simulink model "crs_plant"  (R2026b)
settings: Solver=ode45  StopTime=80  FixedStep=Ts  EnableMultiTasking=on
model workspace (MAT data in the model file):
  Iei = 0.0219914882836
  converter_data = [0  137.465208994  2.232; 0.1  137.065019157  2.075; 0.2  135.864449646  1.975; 0.3  135.664354728  1.846; 0.4  137.565256453  1.72; 0.5  140.366585312  1.564; 0.6  145.268910814  1.409; 0.7  152.872517717  1.254; 0.8  162.9773111  1.096; 0.81  164.27792807  1.08; 0.82  166.178829795  1.061; 0.83  167.979684062  1.043; 0.84  170.080680706  1.028; 0.85  172.781962105  1.012; 0.86  175.383196045  1.002; 0.87  179.585189333  1.002; 0.88  183.587087703  1.001; 0.89  189.890077635  0.998; 0.9  197.693779455  0.999; 0.92  215.902417037  1.001; 0.94  244.515990379  1.002]
  emap = [-40  -44  -49  -53  -57  -61  -65  -70  -74  -78  -82; 215  117  85  66  44  29  10  -2  -13  -22  -32; 245  208  178  148  122  104  85  66  48  33  18; 264  260  241  219  193  167  152  133  119  96  85; 264  279  282  275  260  238  223  208  189  171  152; 267  290  293  297  290  275  260  256  234  212  193; 267  297  305  305  305  301  293  282  267  249  226; 267  301  308  312  319  323  319  316  297  279  253; 267  301  312  319  327  327  327  327  312  293  267; 267  301  312  319  327  334  334  334  319  305  275]
  nevec = [800 1200 1600 2000 2400 2800 3200 3600 4000 4400 4800]
  p0 = 0.07934
  p1 = 0.07934
  thvec = [0; 20; 30; 40; 50; 60; 70; 80; 90; 100]
  vehicledata = [3.23; 40; 0.3; 1; 50; 0]
undefined symbols (not defined in the file): downtab, downth, uptab, upth
settings Model: DataDictionary=crs_plantdic.sldd  SldvGeneratedHarnessModel=TestUnitModel=psui_cruise_control|  Creator=The MathWorks, Inc.  LastModifiedBy=The MathWorks, Inc.
settings DataIOCC: DSMLogging=off  ReturnWorkspaceOutputs=off  SaveFormat=StructureWithTime  SaveOutput=off  SaveTime=off  SignalLogging=off
settings OptimizationCC: BlockReduction=off  ConditionallyExecuteInputs=off  EfficientMapNaN2IntZero=off  LifeSpan=inf  UseDivisionForNetSlopeComputation=on
settings DebuggingCC: AllowSymbolicDim=off  ArithmeticOperatorsInVariantConditions=warning  InheritedTsInSrcMsg=none  SFExecutionAtInitializationDiag=none  SFNoUnconditionalDefaultTransitionDiag=warning  SFUnexpectedBacktrackingDiag=warning  SolverPrmCheckMsg=warning
settings HardwareCC: ProdEndianess=Unspecified  ProdHWDeviceType=32-bit Generic  ProdLargestAtomicFloat=None
settings ModelReferenceCC: PropagateSignalLabelsOutOfModel=off
settings SFSimCC: CustomCodeUndefinedFunction=UseInterfaceOnly  SimUseLocalCustomCode=off
settings RTWCC: DLArmComputeVersion=19.05  RTWUseLocalCustomCode=off
settings CodeAppCC: StateflowObjectComments=on
settings GRTTargetCC: TargetLangStandard=C89/C90 (ANSI)
settings ConfigComp: CovExternalEMLEnable=off  CovHTMLOptions=-sRT=1 -sVT=0 -aTS=1 -bRG=1 -bTC=0 -hTR=0 -nFC=0 -nFD=1 -scm=1 -bcm=1 -xEv=0 -xEM=0  CovMetricSettings=dcm  CovSFcnEnable=off  CovSaveCumulativeToWorkspaceVar=on  CovSaveSingleToWorkspaceVar=on  DVDefectChecker=off  DVDetectActiveLogic=on  DVHarnessSource=Signal Editor  DVSFcnSupport=off  DVTestSuiteOptimization=Auto

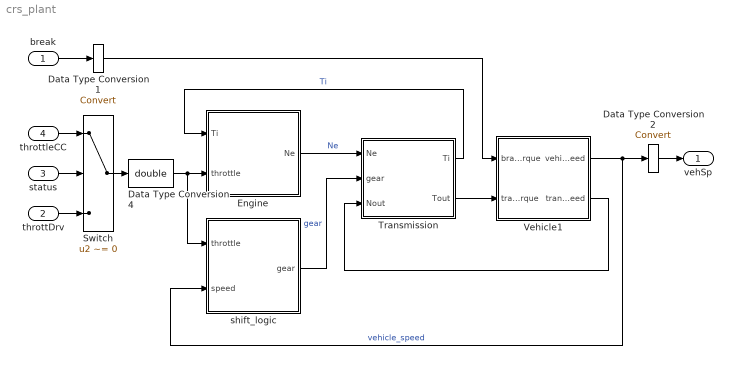
== system crs_plant ==
  break : Inport
  throttDrv : Inport  Port=2
  status : Inport  Port=3  OutDataTypeStr=boolean
  throttleCC : Inport  Port=4
  Data Type Conversion1 : DataTypeConversion  RequirementInfo="{}  %GIDa_0d5f0e68_fee1_41b5_819f_f27f813a37ce"  SaturateOnIntegerOverflow=off  RndMeth=Floor
  Data Type Conversion2 : DataTypeConversion  RequirementInfo="{}  %GIDa_2150bf92_ce46_40fc_a41f_e6b4de8980e5"  SaturateOnIntegerOverflow=off  RndMeth=Floor
  Data Type Conversion4 : DataTypeConversion  RequirementInfo="{}  %GIDa_40e403eb_4293_4261_b76c_ee9daf66d60d"  OutDataTypeStr=double  SaturateOnIntegerOverflow=off  RndMeth=Floor
  Engine : Subsystem
  Switch : Switch  RequirementInfo="{}  %GIDa_4750b5ac_669f_4708_bed6_ecccb1e59b59"  Criteria=u2 ~= 0  SaturateOnIntegerOverflow=off  InputSameDT=off
  Transmission : Subsystem
  Vehicle1 : Subsystem  mask(vehicle model){Rfd=vehicledata(1), rload0=vehicledata(2), rload2=vehicledata(3), Rw=vehicledata(4), Iv=vehicledata(5), N20=vehicledata(6)/vehicledata(4)*vehicledata(1)}
      mask prompts: Rfd "final drive ratio"; rload0 "drag friction at wheels"; rload2 "aerodynamic drag"; Rw "wheel radius"; Iv "vehicle inertia"; N20 "initial transmission output speed"
      mask help: vehicle dynamics: torque input from trans., outputs are input speed (transmission output) and vehicle speed
      mask Display: disp('Vehicle')
  shift_logic : Stateflow chart  TreatAsAtomicUnit=on  mask{TWAIT=2}
      mask prompts: TWAIT "Delay before gear change (tick)"
  vehSp : Outport  VectorParamsAs1DForOutWhenUnconnected=off
  wires:
  Data Type Conversion2/1 -> vehSp/1
  Data Type Conversion1/1 -> Vehicle1/1(brake torque)
  Data Type Conversion4/1 -> shift_logic/1(throttle), Engine/2(throttle)
  shift_logic/1(" gear") -> Transmission/2(gear)  "gear"
  Vehicle1/1(vehicle speed) -> shift_logic/2(speed), Data Type Conversion2/1  "vehicle_speed"
  break/1 -> Data Type Conversion1/1
  throttleCC/1 -> Switch/1
  Engine/1(Ne) -> Transmission/1(Ne)  "Ne"
  Transmission/1(Ti) -> Engine/1(Ti)  "Ti"
  status/1 -> Switch/2
  throttDrv/1 -> Switch/3
  Switch/1 -> Data Type Conversion4/1
  Transmission/2(Tout) -> Vehicle1/2(transmission output torque)
  Vehicle1/2(transmission output speed) -> Transmission/3(Nout)

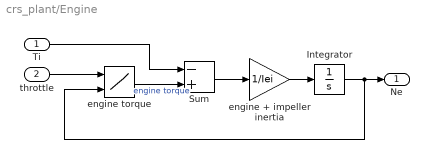
== system crs_plant/Engine ==
  Ti : Inport
  throttle : Inport  Port=2
  Integrator : Integrator  RequirementInfo="{}  %GIDa_40d16765_53ae_4488_8a68_ecbb2df0c680"  InitialCondition=1000  LimitOutput=on  UpperSaturationLimit=6000  LowerSaturationLimit=600  ZeroCross=off
  Sum : Sum  RequirementInfo="{}  %GIDa_1d505b5e_8a80_40cd_8acd_de2326c4a3eb"  Inputs=-+  InputSameDT=on  SaturateOnIntegerOverflow=on  OutDataTypeStr=Inherit: Same as first input
  engine torque : Lookup2D  RequirementInfo="{}  %GIDa_c9ecf741_2e32_444d_a0cd_5ec9da647599"  RowIndex=thvec*0.3  ColumnIndex=nevec  Table=emap  SaturateOnIntegerOverflow=off
  engine + impeller inertia : Gain  RequirementInfo="{}  %GIDa_fbb5ce3c_512e_47cd_b98c_f91ed20f1992"  Gain=1/Iei  SaturateOnIntegerOverflow=on  OutDataTypeStr=Inherit: Same as input  ParamDataTypeStr=Inherit: Same as input
  Ne : Outport  InitialOutput=0  VectorParamsAs1DForOutWhenUnconnected=off
  wires:
  engine torque/1 -> Sum/2  "engine torque"
  engine + impeller inertia/1 -> Integrator/1
  Sum/1 -> engine + impeller inertia/1
  Integrator/1 -> Ne/1, engine torque/2
  throttle/1 -> engine torque/1
  Ti/1 -> Sum/1

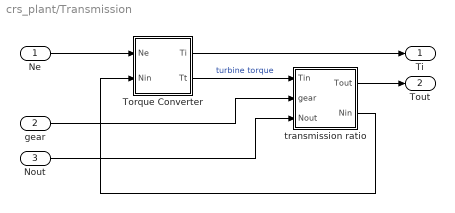
== system crs_plant/Transmission ==
  Ne : Inport
  gear : Inport  Port=2
  Nout : Inport  Port=3
  Torque Converter : Subsystem  mask(torque converter){speedratio=converter_data(:,1), Kfactor=converter_data(:,2), Torkratio=converter_data(:,3)}
      mask prompts: speedratio "speed ratio"; Kfactor "K factor"; Torkratio "torque ratio"
      mask help: torque converter
      mask Help: Torque converter input and output torques are computed as a function of the input and output speeds
      mask Display: plot([cos([90:10:450]*pi/180),.63*cos([90:10:450]*pi/180),.63*cos([90:10:240]*pi/180),cos([240:10:300]*pi/180),.63*cos([300]*pi/180)],[sin([90:10:450]*pi/180),.63*sin([90:10:450]*pi/180)+.1,.63*sin([90:10:240]*pi/180)+.1,sin([240:10:300]*pi/180),.63*sin([300]*pi/180)+.1])
  transmission ratio : Subsystem
  Ti : Outport  VectorParamsAs1DForOutWhenUnconnected=off
  Tout : Outport  Port=2  VectorParamsAs1DForOutWhenUnconnected=off
  wires:
  transmission ratio/1(Tout) -> Tout/1
  Torque Converter/1(Ti) -> Ti/1
  Nout/1 -> transmission ratio/3(Nout)
  gear/1 -> transmission ratio/2(gear)
  Ne/1 -> Torque Converter/1(Ne)
  transmission ratio/2(Nin) -> Torque Converter/2(Nin)
  Torque Converter/2(Tt) -> transmission ratio/1(Tin)  "turbine torque"

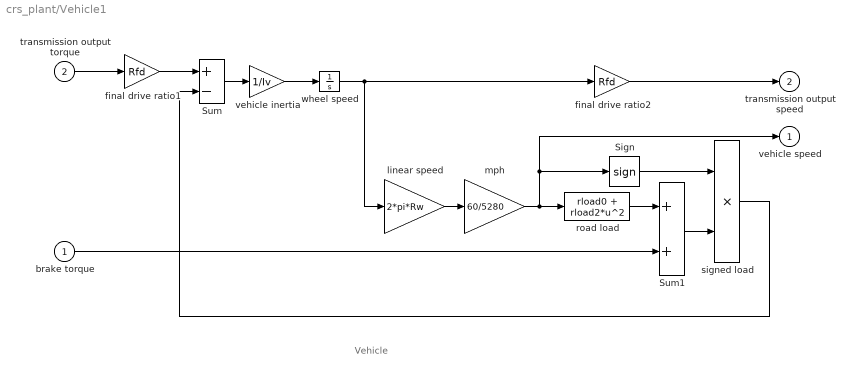
== system crs_plant/Vehicle1 ==
  note: Vehicle
  brake torque : Inport
  transmission output torque : Inport  Port=2
  Sign : Signum
  Sum : Sum  Inputs=+-  InputSameDT=on  SaturateOnIntegerOverflow=on  OutDataTypeStr=Inherit: Same as first input
  Sum1 : Sum  InputSameDT=on  SaturateOnIntegerOverflow=on  OutDataTypeStr=Inherit: Same as first input
  final drive ratio1 : Gain  Gain=Rfd  SaturateOnIntegerOverflow=on  OutDataTypeStr=Inherit: Same as input  ParamDataTypeStr=Inherit: Same as input
  final drive ratio2 : Gain  Gain=Rfd  SaturateOnIntegerOverflow=on  OutDataTypeStr=Inherit: Same as input  ParamDataTypeStr=Inherit: Same as input
  linear speed : Gain  Gain=2*pi*Rw  SaturateOnIntegerOverflow=on  OutDataTypeStr=Inherit: Same as input  ParamDataTypeStr=Inherit: Same as input
  mph : Gain  Gain=60/5280  SaturateOnIntegerOverflow=on  OutDataTypeStr=Inherit: Same as input  ParamDataTypeStr=Inherit: Same as input
  road load : Fcn  Expr=rload0 + rload2*u^2
  signed load : Product  InputSameDT=on  SaturateOnIntegerOverflow=on  OutDataTypeStr=Inherit: Same as first input
  vehicle inertia : Gain  Gain=1/Iv  SaturateOnIntegerOverflow=on  OutDataTypeStr=Inherit: Same as input  ParamDataTypeStr=Inherit: Same as input
  wheel speed : Integrator  InitialCondition=N20/Rfd  ZeroCross=off
  vehicle speed : Outport  VectorParamsAs1DForOutWhenUnconnected=off
  transmission output speed : Outport  Port=2  VectorParamsAs1DForOutWhenUnconnected=off
  wires:
  final drive ratio2/1 -> transmission output speed/1
  brake torque/1 -> Sum1/2
  Sum1/1 -> signed load/2
  road load/1 -> Sum1/1
  Sign/1 -> signed load/1
  signed load/1 -> Sum/2
  transmission output torque/1 -> final drive ratio1/1
  vehicle inertia/1 -> wheel speed/1
  Sum/1 -> vehicle inertia/1
  mph/1 -> vehicle speed/1, Sign/1, road load/1
  linear speed/1 -> mph/1
  wheel speed/1 -> linear speed/1, final drive ratio2/1
  final drive ratio1/1 -> Sum/1

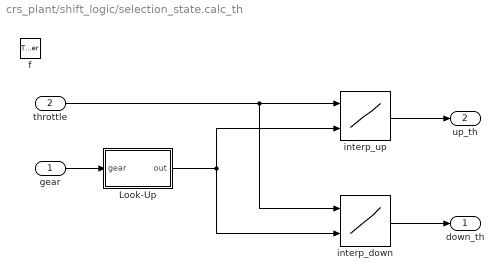
== system crs_plant/shift_logic/selection_state.calc_th ==
  gear : Inport  OutDataTypeStr=Enum: gearType  PortDimensions=1
  throttle : Inport  Port=2  OutDataTypeStr=double  PortDimensions=1
  f : TriggerPort  TriggerType=function-call  VariantControl=Variant
      settings: CopyFcn=Stateflow.SLINSF.SimulinkMan.removeBlockPreDeleteFcn  PreDeleteFcn=Stateflow.SLINSF.SimulinkMan.unsafePredeleteFcn
  Look-Up : MATLAB Function  TreatAsAtomicUnit=on
  interp_down : Lookup_n-D  BreakpointsForDimension1=downth  BreakpointsForDimension2=[1:4]  Table=downtab
      settings: InputPortMap=u0,u1
  interp_up : Lookup_n-D  BreakpointsForDimension1=upth  BreakpointsForDimension2=[1:4]  Table=uptab
      settings: InputPortMap=u0,u1
  down_th : Outport  VectorParamsAs1DForOutWhenUnconnected=off
  up_th : Outport  Port=2  VectorParamsAs1DForOutWhenUnconnected=off
  wires:
  interp_up/1 -> up_th/1
  interp_down/1 -> down_th/1
  throttle/1 -> interp_down/1, interp_up/1
  gear/1 -> Look-Up/1(gear)
  Look-Up/1(out) -> interp_down/2, interp_up/2

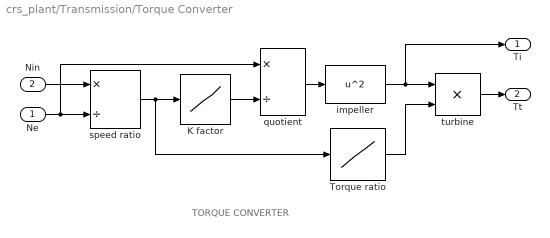
== system crs_plant/Transmission/Torque Converter ==
  note: TORQUE CONVERTER
  Ne : Inport
  Nin : Inport  Port=2
  K factor : Lookup_n-D  NumberOfTableDimensions=1  BreakpointsForDimension1=speedratio  Table=Kfactor  InternalRulePriority=Speed  SaturateOnIntegerOverflow=on
  Torque ratio : Lookup_n-D  NumberOfTableDimensions=1  BreakpointsForDimension1=speedratio  Table=Torkratio  InternalRulePriority=Speed  SaturateOnIntegerOverflow=on
  impeller : Fcn  Expr=u^2
  quotient : Product  Inputs=*/  InputSameDT=on  SaturateOnIntegerOverflow=on  OutDataTypeStr=Inherit: Same as first input
  speed ratio : Product  Inputs=*/  InputSameDT=on  SaturateOnIntegerOverflow=on  OutDataTypeStr=Inherit: Same as first input
  turbine : Product  InputSameDT=on  SaturateOnIntegerOverflow=on  OutDataTypeStr=Inherit: Same as first input
  Ti : Outport  VectorParamsAs1DForOutWhenUnconnected=off
  Tt : Outport  Port=2  VectorParamsAs1DForOutWhenUnconnected=off
  wires:
  Torque ratio/1 -> turbine/2
  quotient/1 -> impeller/1
  K factor/1 -> quotient/2
  speed ratio/1 -> Torque ratio/1, K factor/1
  impeller/1 -> turbine/1, Ti/1
  turbine/1 -> Tt/1
  Ne/1 -> speed ratio/2, quotient/1
  Nin/1 -> speed ratio/1

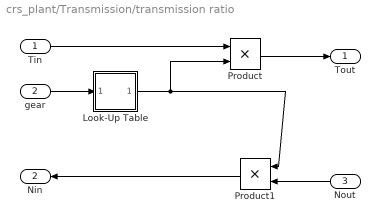
== system crs_plant/Transmission/transmission ratio ==
  Tin : Inport
  gear : Inport  Port=2
  Nout : Inport  Port=3
  Look-Up Table : MATLAB Function  TreatAsAtomicUnit=on
  Product : Product  InputSameDT=on  SaturateOnIntegerOverflow=on  OutDataTypeStr=Inherit: Same as first input
  Product1 : Product  InputSameDT=on  SaturateOnIntegerOverflow=on  OutDataTypeStr=Inherit: Same as first input
  Tout : Outport  VectorParamsAs1DForOutWhenUnconnected=off
  Nin : Outport  Port=2  VectorParamsAs1DForOutWhenUnconnected=off
  wires:
  Look-Up Table/1(out) -> Product1/1, Product/2
  Nout/1 -> Product1/2
  Product1/1 -> Nin/1
  Product/1 -> Tout/1
  gear/1 -> Look-Up Table/1(gear)
  Tin/1 -> Product/1

== stateflow chart crs_plant/shift_logic ==
  settings: updateMethod=DISCRETE  sampleTime=0.04
  state gear_state [parallel]
    settings: executionOrder=1
    state fourth
    state third
    state second
    state first
    (default) -> first
    second -> third [order 1] : UP
    third -> fourth [order 1] : UP
    first -> second : UP
    fourth -> third : DOWN
    third -> second [order 2] : DOWN
    second -> first [order 2] : DOWN
  state selection_state [parallel]
    during: [down_th,up_th] = calc_th(gear,throttle);
    settings: executionOrder=2
    state steady_state
    state upshifting
    state downshifting
    state [down_th,up_th] = calc_th(gear,throttle) [function]
    (default) -> steady_state
    steady_state -> upshifting [order 1] : [speed > up_th]
    steady_state -> downshifting [order 2] : [speed < down_th]
    downshifting -> steady_state [order 1] : after(TWAIT,tick)
        | [speed <= down_th]
        | {send(gear_state.DOWN)}
    downshifting -> steady_state [order 2] : [speed > down_th]
    upshifting -> steady_state [order 1] : after(TWAIT,tick)
        | [speed >= up_th]
        | {send(gear_state.UP)}
    upshifting -> steady_state [order 2] : [speed < up_th]
  data: gear function_input Enum: gearType size=1; throttle function_input double size=1; down_th function_output; up_th function_output; throttle input; speed input double; TWAIT parameter uint8; up_th local double; down_th local double; gear output Enum: gearType
  events: DOWN local EITHER_EDGE_EVENT; UP local EITHER_EDGE_EVENT

== matlab function crs_plant/shift_logic/selection_state.calc_th/Look-Up ==
  data: gear input; out output
function out = fcn(gear)
    %#codegen
    table = [1 2 3 4];
    switch(gear)
        case gearType.fourth;
            out=table(4);        
        case gearType.third;
            out=table(3);
        case gearType.second;
            out=table(2);            
        otherwise; % gearType.first
            out=table(1);
    end
    
end

== matlab function crs_plant/Transmission/transmission ratio/Look-Up Table ==
  data: gear input; out output
function out = fcn(gear)
    %#codegen
    table = [4 3 2 1];
    switch(gear)
        case gearType.fourth;
            out=table(4);        
        case gearType.third;
            out=table(3);            
        case gearType.second;
            out=table(2);
        otherwise; % gearType.first
            out=table(1);
    end
    
end
